simulink model "CircleDiscrete"  (R2025b)
settings: Solver=VariableStepAuto  StartTime=0.0  StopTime=100  RelTol=1e-3  EnableMultiTasking=on
undefined symbols (not defined in the file or in its folder): DiscIntNeverNeededParam, dspblkCoreblockFVToolHelper, gcbh
libraries: simulink x2, slpidlib x2
settings Model: Creator=kkhan  LastModifiedBy=MeisNgan
settings SolverCC: AlgebraicLoopSolver=TrustRegion
settings DataIOCC: ReturnWorkspaceOutputs=off
settings OptimizationCC: LifeSpan=inf
settings DebuggingCC: UnconnectedInputMsg=warning  UnconnectedOutputMsg=warning  UnconnectedLineMsg=warning  SFUnexpectedBacktrackingDiag=warning  SFNoUnconditionalDefaultTransitionDiag=warning  ArithmeticOperatorsInVariantConditions=warning
settings ModelReferenceCC: EnableRefExpFcnMdlSchedulingChecks=on
settings SFSimCC: SimUseLocalCustomCode=off  CustomCodeUndefinedFunction=UseInterfaceOnly
settings RTWCC: RTWUseLocalCustomCode=off  GPUComputeCapability=3.5
settings CodeAppCC: StateflowObjectComments=on
settings GRTTargetCC: TargetLangStandard=C89/C90 (ANSI)
settings ConfigComp: CovMetricSettings=dw  CovSaveCumulativeToWorkspaceVar=on  CovSaveSingleToWorkspaceVar=on  CovExternalEMLEnable=off

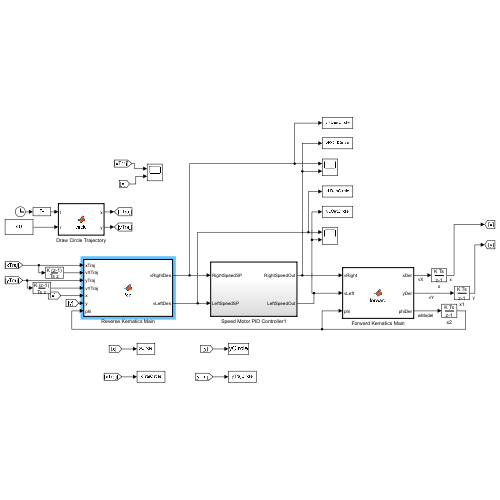
[thumbnail: Simulink's stored preview of the top-level diagram]
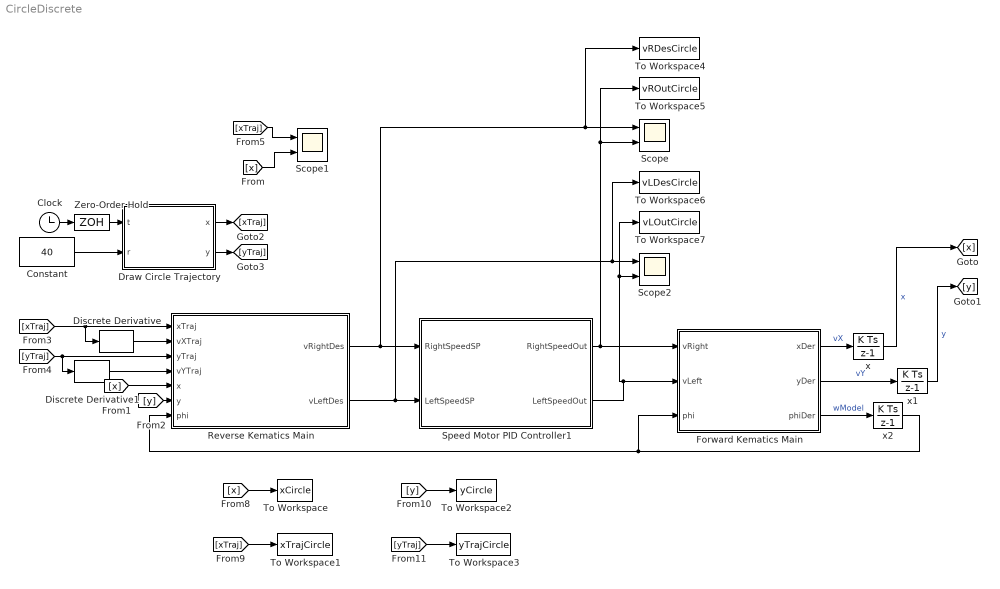
== system CircleDiscrete ==
  Clock : Clock
  Constant : Constant  Value=40
  Discrete Derivative : simulink/Discrete/Discrete Derivative  gainval=1  ICPrevScaledInput=0  OutMin=[]  OutMax=[]  OutDataType=fixdt(1, 16)  OutScaling=2^-10  DoSatur=off
  Discrete Derivative1 : simulink/Discrete/Discrete Derivative  gainval=1  ICPrevScaledInput=0  OutMin=[]  OutMax=[]  OutDataType=fixdt(1, 16)  OutScaling=2^-10  DoSatur=off
  Draw Circle Trajectory : MATLAB Function  TreatAsAtomicUnit=on
  Forward Kematics Main : MATLAB Function  TreatAsAtomicUnit=on
  Reverse Kematics Main : MATLAB Function  TreatAsAtomicUnit=on
  Scope : Scope  NumInputPorts=2
      settings: ActiveDisplayYMinimum=-33.960779793631076  ActiveDisplayYMaximum=397.19925208731138  DataLoggingSaveFormat=Array
  Scope1 : Scope  NumInputPorts=2
      settings: ActiveDisplayYMinimum=38.4522930792872  ActiveDisplayYMaximum=40.425845327430132  DataLoggingVariableName=ScopeData2  DataLoggingSaveFormat=Array
  Scope2 : Scope  NumInputPorts=2
      settings: DataLoggingVariableName=ScopeData3  DataLoggingSaveFormat=Array
  Speed Motor PID Controller1 : Subsystem  TreatAsAtomicUnit=on
  To Workspace : ToWorkspace  VariableName=xCircle  SaveFormat=Timeseries  SampleTime=-1
      settings: Decimation=2
  To Workspace1 : ToWorkspace  VariableName=xTrajCircle  SaveFormat=Timeseries  SampleTime=-1
      settings: Decimation=2
  To Workspace2 : ToWorkspace  VariableName=yCircle  SaveFormat=Timeseries  SampleTime=-1
      settings: Decimation=2
  To Workspace3 : ToWorkspace  VariableName=yTrajCircle  SaveFormat=Timeseries  SampleTime=-1
      settings: Decimation=2
  To Workspace4 : ToWorkspace  VariableName=vRDesCircle  SaveFormat=Timeseries  SampleTime=-1
      settings: Decimation=2
  To Workspace5 : ToWorkspace  VariableName=vROutCircle  SaveFormat=Timeseries  SampleTime=-1
      settings: Decimation=2
  To Workspace6 : ToWorkspace  VariableName=vLDesCircle  SaveFormat=Timeseries  SampleTime=-1
      settings: Decimation=2
  To Workspace7 : ToWorkspace  VariableName=vLOutCircle  SaveFormat=Timeseries  SampleTime=-1
      settings: Decimation=2
  Zero-Order Hold : ZeroOrderHold  SampleTime=0.02
  x : DiscreteIntegrator  SampleTime=0.02  ICPrevOutput=DiscIntNeverNeededParam  ICPrevScaledInput=DiscIntNeverNeededParam
  x1 : DiscreteIntegrator  SampleTime=0.02  ICPrevOutput=DiscIntNeverNeededParam  ICPrevScaledInput=DiscIntNeverNeededParam
  x2 : DiscreteIntegrator  SampleTime=0.02  ICPrevOutput=DiscIntNeverNeededParam  ICPrevScaledInput=DiscIntNeverNeededParam
  wires:
  Speed Motor PID Controller1/2(LeftSpeedOut) -> Forward Kematics Main/2(vLeft), To Workspace7/1, Scope2/2
  Forward Kematics Main/1(xDer) -> x/1  "vX"
  Forward Kematics Main/2(yDer) -> x1/1  "vY"
  x/1 -> [x]  "x"
  x1/1 -> [y]  "y"
  Forward Kematics Main/3(phiDer) -> x2/1  "wModel"
  x2/1 -> Reverse Kematics Main/7(phi), Forward Kematics Main/3(phi)
  Discrete Derivative/1 -> Reverse Kematics Main/2(vXTraj)
  Discrete Derivative1/1 -> Reverse Kematics Main/4(vYTraj)
  [x] -> Scope1/2
  [x] -> Reverse Kematics Main/5(x)
  [y] -> Reverse Kematics Main/6(y)
  [xTraj] -> Discrete Derivative/1, Reverse Kematics Main/1(xTraj)
  [yTraj] -> Discrete Derivative1/1, Reverse Kematics Main/3(yTraj)
  [xTraj] -> Scope1/1
  Draw Circle Trajectory/1(x) -> [xTraj]
  Draw Circle Trajectory/2(y) -> [yTraj]
  [x] -> To Workspace/1
  [xTraj] -> To Workspace1/1
  [y] -> To Workspace2/1
  [yTraj] -> To Workspace3/1
  Reverse Kematics Main/1(vRightDes) -> Speed Motor PID Controller1/1(RightSpeedSP), To Workspace4/1, Scope/1
  Speed Motor PID Controller1/1(RightSpeedOut) -> Forward Kematics Main/1(vRight), Scope/2, To Workspace5/1
  Reverse Kematics Main/2(vLeftDes) -> Speed Motor PID Controller1/2(LeftSpeedSP), To Workspace6/1, Scope2/1
  Constant/1 -> Draw Circle Trajectory/2(r)
  Clock/1 -> Zero-Order Hold/1
  Zero-Order Hold/1 -> Draw Circle Trajectory/1(t)

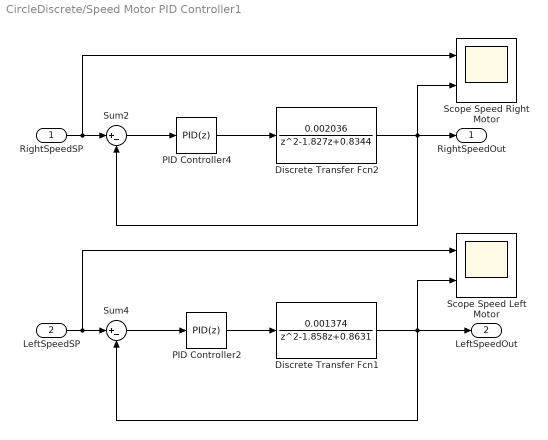
== system CircleDiscrete/Speed Motor PID Controller1 ==
  RightSpeedSP : Inport
  LeftSpeedSP : Inport  Port=2
  Discrete Transfer Fcn1 : DiscreteTransferFcn  Numerator=[0.001374]  Denominator=[1 -1.858 0.8631]  SampleTime=0.02
  Discrete Transfer Fcn2 : DiscreteTransferFcn  LoadFcn=dspblkCoreblockFVToolHelper(gcbh,'load');  Numerator=[0.002036]  Denominator=[1 -1.827 0.8344]  SampleTime=0.02
      settings: CopyFcn=dspblkCoreblockFVToolHelper(gcbh,'copy');  DeleteFcn=dspblkCoreblockFVToolHelper(gcbh,'close');  ModelCloseFcn=dspblkCoreblockFVToolHelper(gcbh,'close');  PreSaveFcn=dspblkCoreblockFVToolHelper(gcbh,'presave');  PostSaveFcn=dspblkCoreblockFVToolHelper(gcbh,'postsave');  CloseFcn=dspblkCoreblockFVToolHelper(gcbh,'close');
  PID Controller2 : slpidlib/PID Controller  Controller=PID  Form=Parallel  TimeDomain=Discrete-time  UseExternalTs=off  SampleTime=0.02  IntegratorMethod=Forward Euler  FilterMethod=Forward Euler  ControllerParametersSource=internal  P=21.0909852919714  I=43.5478218388463  UseKiTs=off  D=2.15960697462874  UseExternalDerivativeSource=off  N=26.7883535297543  UseFilter=on  TunerSelectOption=Transfer Function Based (PID Tuner App)  InitialConditionSource=internal  InitialConditionForIntegrator=0  InitialConditionForFilter=0  DifferentiatorICPrevScaledInput=0  ExternalReset=none  TrackingMode=off  Kt=1  LimitOutput=off  SatLimitsSource=internal  UpperSaturationLimit=inf  LowerSaturationLimit=-inf  LinearizeAsGain=on  AntiWindupMode=none  Kb=1  LimitIntegrator=off  UpperIntegratorSaturationLimit=inf  LowerIntegratorSaturationLimit=-inf  POutMin=[]  POutMax=[]  IOutMin=[]  IOutMax=[]  DOutMin=[]  DOutMax=[]  NOutMin=[]  NOutMax=[]  SumOutMin=[]  SumOutMax=[]  SaturationOutMin=[]  SaturationOutMax=[]  PParamMin=[]  PParamMax=[]  IParamMin=[]  IParamMax=[]  DParamMin=[]  DParamMax=[]  NParamMin=[]  NParamMax=[]  KbParamMin=[]  KbParamMax=[]  KtParamMin=[]  KtParamMax=[]  KbOutMin=[]  KbOutMax=[]  KtOutMin=[]  KtOutMax=[]  IntegratorOutMin=[]  IntegratorOutMax=[]  FilterOutMin=[]  FilterOutMax=[]  SumI1OutMin=[]  SumI1OutMax=[]  SumI2OutMin=[]  SumI2OutMax=[]  SumI3OutMin=[]  SumI3OutMax=[]  SumI4OutMin=[]  SumI4OutMax=[]  SumDOutMin=[]  SumDOutMax=[]  DifferentiatorOutMin=[]  DifferentiatorOutMax=[]  FilterDiffOutCoefMin=[]  FilterDiffOutCoefMax=[]  ReciprocalOutMin=[]  ReciprocalOutMax=[]  SumDenOutMin=[]  SumDenOutMax=[]  SumNumOutMin=[]  SumNumOutMax=[]  DivideOutMin=[]  DivideOutMax=[]  UdiffTsProdOutMin=[]  UdiffTsProdOutMax=[]  NTsProdOutMin=[]  NTsProdOutMax=[]  UintegralTsProdOutMin=[]  UintegralTsProdOutMax=[]  UngainTsProdOutMin=[]  UngainTsProdOutMax=[]  ClampingZeroOutDataTypeStr=Inherit: Inherit via back propagation  ClampingZeroOutMin=[]  ClampingZeroOutMax=[]  FilterDenConstantOutDataTypeStr=Inherit: Inherit via back propagation  FilterDenConstantOutMin=[]  FilterDenConstantOutMax=[]  PCopyOutDataTypeStr=Inherit: Inherit via back propagation  PCopyOutMin=[]  PCopyOutMax=[]  NCopyOutDataTypeStr=Inherit: Inherit via back propagation  NCopyOutMin=[]  NCopyOutMax=[]  IntegratorContinuousStateAttributes=''  IntegratorStateMustResolveToSignalObject=off  IntegratorRTWStateStorageClass=Auto  FilterContinuousStateAttributes=''  FilterStateMustResolveToSignalObject=off  FilterRTWStateStorageClass=Auto  ParallelPVariant=InternalParameters  IdealPVariant=Disabled  IVariant=InternalParameters  DVariant=InternalParameters  IntegratorVariant=Discrete  SatVariant=Disabled  AWVariant=Passthrough  PCopyVariant=Disabled  TRVariant=Disabled  FdbkBlocksVariant=Forward  IdealPFdbkVariant=Disabled  SatFdbkVariant=Disabled  DerivativeFilterVariant=ForwardEulerFilter  NVariant=InternalParameters  NCopyVariant=Disabled  FilterICVariant=InternalICsFilter  IntegratorICVariant=InternalICs  ExternalResetVariant=Disabled  TRSumVariant=Passthrough  SumFdbkVariant=Disabled  SumVariant=Sum_PID  TsampFilterVariant=InternalTs  TsampNgainVariant=Passthrough  TsampIntegralVariant=Disabled_SignalSpec  ExternalSaturationOutDataTypeStr=Inherit: Same as second input  DerivativeSourceVariant=ErrorSignal  PreIntVariant=InternalPreInt
  PID Controller4 : slpidlib/PID Controller  Controller=PID  Form=Parallel  TimeDomain=Discrete-time  UseExternalTs=off  SampleTime=0.02  IntegratorMethod=Forward Euler  FilterMethod=Forward Euler  ControllerParametersSource=internal  P=16.8217157087944  I=42.6084644082369  UseKiTs=off  D=1.35986407955998  UseExternalDerivativeSource=off  N=26.7883535297543  UseFilter=on  TunerSelectOption=Transfer Function Based (PID Tuner App)  InitialConditionSource=internal  InitialConditionForIntegrator=0  InitialConditionForFilter=0  DifferentiatorICPrevScaledInput=0  ExternalReset=none  TrackingMode=off  Kt=1  LimitOutput=off  SatLimitsSource=internal  UpperSaturationLimit=inf  LowerSaturationLimit=-inf  LinearizeAsGain=on  AntiWindupMode=none  Kb=1  LimitIntegrator=off  UpperIntegratorSaturationLimit=inf  LowerIntegratorSaturationLimit=-inf  POutMin=[]  POutMax=[]  IOutMin=[]  IOutMax=[]  DOutMin=[]  DOutMax=[]  NOutMin=[]  NOutMax=[]  SumOutMin=[]  SumOutMax=[]  SaturationOutMin=[]  SaturationOutMax=[]  PParamMin=[]  PParamMax=[]  IParamMin=[]  IParamMax=[]  DParamMin=[]  DParamMax=[]  NParamMin=[]  NParamMax=[]  KbParamMin=[]  KbParamMax=[]  KtParamMin=[]  KtParamMax=[]  KbOutMin=[]  KbOutMax=[]  KtOutMin=[]  KtOutMax=[]  IntegratorOutMin=[]  IntegratorOutMax=[]  FilterOutMin=[]  FilterOutMax=[]  SumI1OutMin=[]  SumI1OutMax=[]  SumI2OutMin=[]  SumI2OutMax=[]  SumI3OutMin=[]  SumI3OutMax=[]  SumI4OutMin=[]  SumI4OutMax=[]  SumDOutMin=[]  SumDOutMax=[]  DifferentiatorOutMin=[]  DifferentiatorOutMax=[]  FilterDiffOutCoefMin=[]  FilterDiffOutCoefMax=[]  ReciprocalOutMin=[]  ReciprocalOutMax=[]  SumDenOutMin=[]  SumDenOutMax=[]  SumNumOutMin=[]  SumNumOutMax=[]  DivideOutMin=[]  DivideOutMax=[]  UdiffTsProdOutMin=[]  UdiffTsProdOutMax=[]  NTsProdOutMin=[]  NTsProdOutMax=[]  UintegralTsProdOutMin=[]  UintegralTsProdOutMax=[]  UngainTsProdOutMin=[]  UngainTsProdOutMax=[]  ClampingZeroOutDataTypeStr=Inherit: Inherit via back propagation  ClampingZeroOutMin=[]  ClampingZeroOutMax=[]  FilterDenConstantOutDataTypeStr=Inherit: Inherit via back propagation  FilterDenConstantOutMin=[]  FilterDenConstantOutMax=[]  PCopyOutDataTypeStr=Inherit: Inherit via back propagation  PCopyOutMin=[]  PCopyOutMax=[]  NCopyOutDataTypeStr=Inherit: Inherit via back propagation  NCopyOutMin=[]  NCopyOutMax=[]  IntegratorContinuousStateAttributes=''  IntegratorStateMustResolveToSignalObject=off  IntegratorRTWStateStorageClass=Auto  FilterContinuousStateAttributes=''  FilterStateMustResolveToSignalObject=off  FilterRTWStateStorageClass=Auto  ParallelPVariant=InternalParameters  IdealPVariant=Disabled  IVariant=InternalParameters  DVariant=InternalParameters  IntegratorVariant=Discrete  SatVariant=Disabled  AWVariant=Passthrough  PCopyVariant=Disabled  TRVariant=Disabled  FdbkBlocksVariant=Forward  IdealPFdbkVariant=Disabled  SatFdbkVariant=Disabled  DerivativeFilterVariant=ForwardEulerFilter  NVariant=InternalParameters  NCopyVariant=Disabled  FilterICVariant=InternalICsFilter  IntegratorICVariant=InternalICs  ExternalResetVariant=Disabled  TRSumVariant=Passthrough  SumFdbkVariant=Disabled  SumVariant=Sum_PID  TsampFilterVariant=InternalTs  TsampNgainVariant=Passthrough  TsampIntegralVariant=Disabled_SignalSpec  ExternalSaturationOutDataTypeStr=Inherit: Same as second input  DerivativeSourceVariant=ErrorSignal  PreIntVariant=InternalPreInt
  Scope Speed Left Motor : Scope  NumInputPorts=2
      settings: ActiveDisplayYMinimum=-8.74589  ActiveDisplayYMaximum=5.70257
  Scope Speed Right Motor : Scope  NumInputPorts=2
      settings: ActiveDisplayYMinimum=-2.00121  ActiveDisplayYMaximum=18.01087
  Sum2 : Sum  Inputs=|+-
  Sum4 : Sum  Inputs=|+-
  RightSpeedOut : Outport
  LeftSpeedOut : Outport  Port=2
  wires:
  PID Controller2/1 -> Discrete Transfer Fcn1/1
  Sum4/1 -> PID Controller2/1
  Discrete Transfer Fcn1/1 -> Sum4/2, LeftSpeedOut/1, Scope Speed Left Motor/2
  LeftSpeedSP/1 -> Sum4/1, Scope Speed Left Motor/1
  PID Controller4/1 -> Discrete Transfer Fcn2/1
  Sum2/1 -> PID Controller4/1
  Discrete Transfer Fcn2/1 -> Sum2/2, RightSpeedOut/1, Scope Speed Right Motor/2
  RightSpeedSP/1 -> Sum2/1, Scope Speed Right Motor/1

== matlab function CircleDiscrete/Forward Kematics Main ==
  data: vRight input; xDer output; vLeft input; yDer output; phiDer output; phi input
function [xDer,yDer,phiDer] = forward(vRight, vLeft, phi)
%#codegen
%Thong so mo hinh
lWheel = 8;
c = 4;
%Input la van toc [cm/s]
vModel = (vRight + vLeft)/2;
%Van toc goc nay la cua mo hinh
wModel = (vRight - vLeft)/(2*lWheel);

vectorMatrix = [cos(phi), -c*sin(phi);
            sin(phi), c*cos(phi);
            0, 1];
velMatrix = [vModel;wModel];

posMatrix = vectorMatrix*velMatrix;

xDer = posMatrix(1);
yDer = posMatrix(2);
phiDer = posMatrix(3);

== matlab function CircleDiscrete/Draw Circle Trajectory ==
  data: x output; t input; y output; r input
function [x,y] = circle(t,r)
%#codegen
w = pi/16;
x = r*cos(w*t);
y = r*sin(w*t);

== matlab function CircleDiscrete/Reverse Kematics Main ==
  data: xTraj input; vXTraj input; yTraj input; vYTraj input; x input; y input; vRightDes output; vLeftDes output; phi input
function [vRightDes,vLeftDes] = fcn(xTraj,vXTraj,yTraj,vYTraj,x,y,phi)
%#codegen
L = 16;
c = 4;
lx = 22;
ly = 18;
kx = 1;
ky = 1;
%Input la toa do x, y
%Tu do dao ham se ra van toc dai [cm/s]
stateMatrix = [cos(phi), sin(phi);
               (-1/c)*sin(phi), (1/c)*cos(phi)];
velMatrix = stateMatrix*[vXTraj + lx*tanh((kx/lx)*(xTraj-x));
                         vYTraj + ly*tanh((ky/ly)*(yTraj-y))];

M = [1, L/2; 1, -L/2];
velRLMatrix = M*velMatrix;

vRightDes = velRLMatrix(1);
vLeftDes = velRLMatrix(2);
